simulink model "ARDroneControl"  (R2024a)
settings: Solver=ode1  StartTime=0.0  StopTime=inf  FixedStep=sampleTime  RelTol=1e-3  EnableMultiTasking=on
InitFcn:
  | run('/Users/usuario/Desktop/MEAer/TFM/End-end system/ARDroneSimulinkDevKit_V1.1 hover/wifiControl/DroneStream_tracking_init.m')
undefined symbols (not defined in the file): sampleTime, Standard_Devices, UDP_Protocol
libraries: sldrtlib x3, dspnetwork x3, aerolibanimutils x1
settings Model: ExtModeTrigDuration=100000  Creator=Paul  LastModifiedBy=usuario
settings SolverCC: AlgebraicLoopSolver=TrustRegion  AutoInsertRateTranBlk=on
settings DataIOCC: LimitDataPoints=on  SaveFormat=StructureWithTime  SignalLoggingSaveFormat=ModelDataLogs  ReturnWorkspaceOutputs=off  TimeSaveName=time
settings OptimizationCC: BlockReduction=off  OptimizeBlockIOStorage=off  BufferReuse=off  GlobalBufferReuse=off  ExpressionFolding=off  ExpressionDepthLimit=2147483647  LocalBlockOutputs=off  InitFltsAndDblsToZero=on  OptimizeDataStoreBuffers=off  BusAssignmentInplaceUpdate=off
settings DebuggingCC: UnderspecifiedInitializationDetection=Classic  MergeDetectMultiDrivingBlocksExec=none  SolverPrmCheckMsg=warning  FcnCallInpInsideContextMsg=warning  UnconnectedInputMsg=warning  UnconnectedOutputMsg=warning  UnconnectedLineMsg=warning  StateNameClashWarn=warning  SFUnexpectedBacktrackingDiag=warning  SFNoUnconditionalDefaultTransitionDiag=warning  SFExecutionAtInitializationDiag=none  ArithmeticOperatorsInVariantConditions=warning
settings HardwareCC: ProdBitPerLong=64  ProdHWDeviceType=Intel->x86-64 (Mac OS X)
settings ModelReferenceCC: EnableRefExpFcnMdlSchedulingChecks=on  PropagateSignalLabelsOutOfModel=off
settings SFSimCC: SimUseLocalCustomCode=off  CustomCodeUndefinedFunction=UseInterfaceOnly
settings RTWCC: Description=Simulink Desktop Real-Time  SystemTargetFile=sldrt.tlc  TemplateMakefile=sldrt.tmf  RTWUseLocalCustomCode=off  RTWCompilerOptimization=on  GPUComputeCapability=3.5
settings CodeAppCC: MaxIdLength=95  StateflowObjectComments=on
settings SimulinkDesktopRealTimeCC: TargetPreCompLibLocation=/Applications/MATLAB_R2017b.app/toolbox/sldrt/lib/maci64  TargetLangStandard=C89/C90 (ANSI)
settings ConfigComp: CovMetricSettings=dw  CovSaveCumulativeToWorkspaceVar=on  CovSaveSingleToWorkspaceVar=on  CovExternalEMLEnable=off

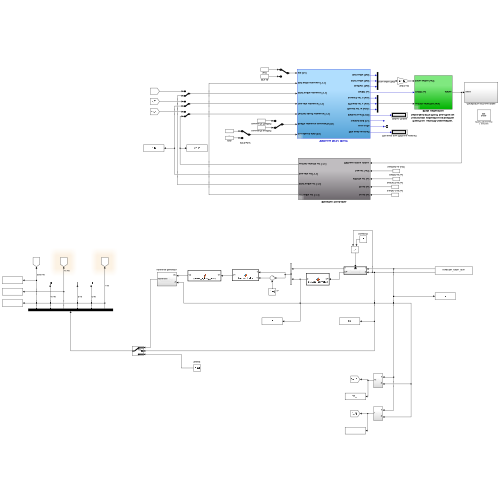
[thumbnail: Simulink's stored preview of the top-level diagram]
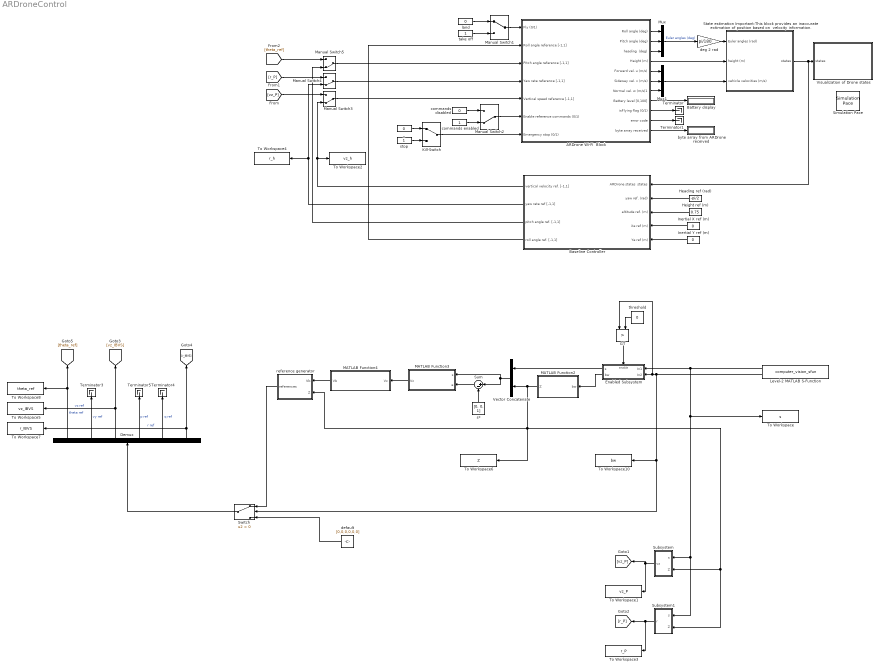
== system ARDroneControl ==
  ARDrone Wi-Fi  Block : Subsystem  AncestorBlock="ARBlocks/ARDrone Wi-Fi  Block"
  Baseline Controller : Subsystem  AncestorBlock=ARBlocks/Baseline Controller
  Battery display : Display
  Demux : Demux  Outputs=6
  Enabled Subsystem : Subsystem  TreatAsAtomicUnit=on
  GT : RelationalOperator  Operator=>  OutDataTypeStr=boolean  RndMeth=Simplest  InputSameDT=off
  Heading ref (rad) : Constant  Value=-pi/2
  Height ref (m) : Constant  Value=0.75
  Inertial X ref (m) : Constant  Value=0
  Inertial Y ref (m) : Constant  Value=0
  Kill-Switch : ManualSwitch
  Level-2 MATLAB S-Function : M-S-Function  FunctionName=computer_vision_sfun
  MATLAB Function2 : MATLAB Function  TreatAsAtomicUnit=on
  MATLAB Function3 : MATLAB Function  TreatAsAtomicUnit=on
  MATLAB Function4 : MATLAB Function  TreatAsAtomicUnit=on
  Manual Switch1 : ManualSwitch
  Manual Switch{2..5} (4 alike) : ManualSwitch  CurrentSetting=0
  Mux : Mux  Inputs=3
  Mux1 : Mux  Inputs=3
  Simulation Pace : aerolibanimutils/Simulation Pace  SimulationPace=1  SleepMode=MATLAB Thread  OutputPaceError=off  SampleTime=sampleTime
  "State estimation Important:This block provides an inaccurate extimation of position based on  velocity information. " : Subsystem  AncestorBlock=|
      | ARBlocks/Position estimation
      | Important:This block provides an 
      | inaccurate extimation of position 
      | based on  velocity information.
  Subsystem : Subsystem
  Subsystem1 : Subsystem
  Sum : Sum  Inputs=|+-
  Switch : Switch  Criteria=u2 > Threshold  SaturateOnIntegerOverflow=off  InputSameDT=off
  Terminator{,1,3..5} (5 alike) : Terminator
  To Workspace : ToWorkspace  VariableName=s  SaveFormat=Timeseries  SampleTime=-1
  To Workspace1 : ToWorkspace  VariableName=vz_P  SaveFormat=Timeseries  SampleTime=-1
  To Workspace10 : ToWorkspace  VariableName=bw  SaveFormat=Timeseries  SampleTime=-1
  To Workspace2 : ToWorkspace  VariableName=vz_h  SaveFormat=Timeseries  SampleTime=-1
  To Workspace3 : ToWorkspace  VariableName=r_P  SaveFormat=Timeseries  SampleTime=-1
  To Workspace4 : ToWorkspace  VariableName=r_h  SaveFormat=Timeseries  SampleTime=-1
  To Workspace5 : ToWorkspace  VariableName=vz_IBVS  SaveFormat=Timeseries  SampleTime=-1
  To Workspace6 : ToWorkspace  VariableName=Z  SaveFormat=Timeseries  SampleTime=-1
  To Workspace7 : ToWorkspace  VariableName=r_IBVS  SaveFormat=Timeseries  SampleTime=-1
  To Workspace8 : ToWorkspace  VariableName=theta_ref  SaveFormat=Timeseries  SampleTime=-1
  Vector Concatenate : Concatenate
  Visualization of Drone states : Subsystem
  _ : Constant  Value=0
  "byte array from ARDrone received " : Display
  commands disabled : Constant  Value=0
  commands enabled : Constant
  default : Constant  Value=[0,0,0,0,0,0]
  deg 2 rad : Gain  Gain=pi/180
  land : Constant  Value=0
  reference generator : Subsystem
  s* : Constant  Value=[0, 0, 1]
  stop : Constant
  take off : Constant
  threshold : Constant  Value=0
  wires:
  _/1 -> Kill-Switch/1
  stop/1 -> Kill-Switch/2
  land/1 -> Manual Switch1/1
  take off/1 -> Manual Switch1/2
  commands disabled/1 -> Manual Switch2/1
  commands enabled/1 -> Manual Switch2/2
  Manual Switch1/1 -> ARDrone Wi-Fi  Block/1(Fly (0/1))
  Manual Switch2/1 -> ARDrone Wi-Fi  Block/6(Enable reference commands (0/1))
  Kill-Switch/1 -> ARDrone Wi-Fi  Block/7(Emergency stop (0/1))
  ARDrone Wi-Fi  Block/1(Roll angle (deg)) -> Mux/1
  ARDrone Wi-Fi  Block/2(Pitch angle (deg)) -> Mux/2
  ARDrone Wi-Fi  Block/5(Forward vel. u (m/s)) -> Mux1/1
  ARDrone Wi-Fi  Block/6(Sideway vel. v (m/s)) -> Mux1/2
  ARDrone Wi-Fi  Block/7(Normal vel. w (m/s)1) -> Mux1/3
  Mux/1 -> deg 2 rad/1  "Euler angles (deg)"
  ARDrone Wi-Fi  Block/8(Battery level [0,100]) -> Battery display/1
  "State estimation Important:This block provides an inaccurate extimation of position based on  velocity information. "/1(states) -> Baseline Controller/1("ARDrone states  states "), Visualization of Drone states/1(states)
  deg 2 rad/1 -> "State estimation Important:This block provides an inaccurate extimation of position based on  velocity information. "/1(Euler angles (rad))
  Mux1/1 -> "State estimation Important:This block provides an inaccurate extimation of position based on  velocity information. "/3(vehicle velocities (m/s))
  ARDrone Wi-Fi  Block/3(heading  (deg)) -> Mux/3
  ARDrone Wi-Fi  Block/9(isFlying flag (0/1)) -> Terminator/1
  ARDrone Wi-Fi  Block/10(error code) -> Terminator1/1
  ARDrone Wi-Fi  Block/11(byte array received) -> "byte array from ARDrone received "/1
  ARDrone Wi-Fi  Block/4(Height (m)) -> "State estimation Important:This block provides an inaccurate extimation of position based on  velocity information. "/2(height (m))
  Heading ref (rad)/1 -> Baseline Controller/2(yaw ref. (rad))
  Inertial Y ref (m)/1 -> Baseline Controller/5(Ye ref (m))
  Inertial X ref (m)/1 -> Baseline Controller/4(Xe ref (m))
  Baseline Controller/4(roll angle ref. [-1,1]) -> ARDrone Wi-Fi  Block/2(Roll angle reference [-1,1])
  Height ref (m)/1 -> Baseline Controller/3(altitude ref. (m))
  s*/1 -> Sum/2
  Demux/4 -> Terminator5/1  "p ref"
  Demux/2 -> Terminator3/1  "vy ref"
  Sum/1 -> MATLAB Function3/2(e)
  Level-2 MATLAB S-Function/1 -> Subsystem1/1(s), Subsystem/1(s), To Workspace/1, Enabled Subsystem/1(In1)
  MATLAB Function2/1(Z) -> reference generator/2(Z), Subsystem/2(Z), Subsystem1/2(Z), To Workspace6/1, Vector Concatenate/2
  MATLAB Function3/1(Vc) -> MATLAB Function4/1(Vc)
  Demux/5 -> Terminator4/1  "q ref"
  Demux/3 -> To Workspace5/1, [vz_IBVS]  "vz ref"
  Demux/6 -> [r_IBVS], To Workspace7/1  "r ref"
  [vz_P] -> Manual Switch3/1
  [r_P] -> Manual Switch4/1
  Manual Switch4/1 -> ARDrone Wi-Fi  Block/4(Yaw rate reference [-1,1])
  Manual Switch3/1 -> ARDrone Wi-Fi  Block/5(Vertical speed reference [-1,1])
  Baseline Controller/1(vertical velocity ref. [-1,1]) -> Manual Switch3/2, To Workspace2/1
  Baseline Controller/2(yaw rate ref [-1,1]) -> Manual Switch4/2, To Workspace4/1
  Subsystem/1(vz) -> [vz_P], To Workspace1/1
  Subsystem1/1(r) -> To Workspace3/1, [r_P]
  Level-2 MATLAB S-Function/2 -> Enabled Subsystem/2(In2), GT/1, Switch/2, To Workspace10/1
  GT/1 -> Enabled Subsystem/Enable
  threshold/1 -> GT/2
  Switch/1 -> Demux/1
  default/1 -> Switch/3
  Enabled Subsystem/1(s) -> Vector Concatenate/1
  Enabled Subsystem/2(bw) -> MATLAB Function2/1(bw)
  Demux/1 -> To Workspace8/1, [theta_ref]  "theta ref"
  Manual Switch5/1 -> ARDrone Wi-Fi  Block/3(Pitch angle reference [-1,1])
  [theta_ref] -> Manual Switch5/1
  Baseline Controller/3(pitch angle ref. [-1,1]) -> Manual Switch5/2
  MATLAB Function4/1(Vb) -> reference generator/1(Vb)
  reference generator/1(references) -> Switch/1
  Vector Concatenate/1 -> Sum/1, MATLAB Function3/1(s)

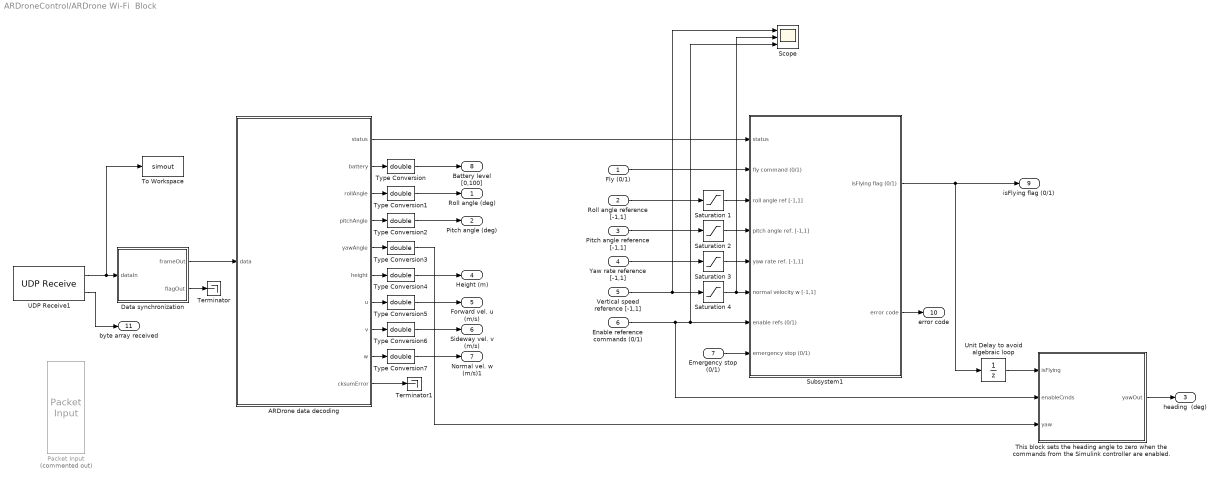
== system ARDroneControl/ARDrone Wi-Fi  Block ==
  Fly (0/1) : Inport
  Roll angle reference [-1,1] : Inport  Port=2
  Pitch angle reference [-1,1] : Inport  Port=3
  Yaw rate reference [-1,1] : Inport  Port=4
  Vertical speed reference [-1,1] : Inport  Port=5
  Enable reference commands (0/1) : Inport  Port=6
  Emergency stop (0/1) : Inport  Port=7
  ARDrone data decoding : MATLAB Function  TreatAsAtomicUnit=on
  "Data synchronization " : MATLAB Function  TreatAsAtomicUnit=on
  Packet Input : sldrtlib/Packet Input  Commented=on  SampleTime=sampleTime  MaxMissedTicks=100  ShowMissedTicks=off  YieldWhenWaiting=off  DrvName=Standard_Devices/UDP_Protocol  DrvAddress=5554  DrvOptions=[3232235777 5554]  PacketSize=500  DataTypes='500*uint8'  ShowReady=on  ShowError=off  PacketID=1  ByteOrder=1  ShowTimestamp=off
      settings: AttributesFormatString=UDP Protocol [5554]
  Saturation 1 : Saturate  UpperLimit=1  LowerLimit=-1
  Saturation 2 : Saturate  UpperLimit=1  LowerLimit=-1
  Saturation 3 : Saturate  UpperLimit=1  LowerLimit=-1
  Saturation 4 : Saturate  UpperLimit=1.5  LowerLimit=-1.5
  Scope : Scope  NumInputPorts=3
  Subsystem1 : Subsystem
  Terminator : Terminator
  Terminator1 : Terminator
  "This block sets the heading angle to zero when the commands from the Simulink controller are enabled. " : MATLAB Function  TreatAsAtomicUnit=on
  To Workspace : ToWorkspace  VariableName=simout  SampleTime=-1
  Type Conversion{,1..7} (8 alike) : DataTypeConversion  OutDataTypeStr=double  SaturateOnIntegerOverflow=off  RndMeth=Floor
  UDP Receive1 : dspnetwork/UDP Receive  localURL='0.0.0.0'  localPort=5554  remoteURL='192.168.1.1'  remotePort=-1  recvBufferSize=8192  dims=500  signalDatatype=uint8  isComplex=off  isVarSize=off  showBlockingTime=off  blockingTime=0  sampletime=sampleTime  blockPlatform=[]
  Unit Delay to avoid algebraic loop : UnitDelay  SampleTime=-1  HasFrameUpgradeWarning=on
  Roll angle (deg) : Outport  VectorParamsAs1DForOutWhenUnconnected=off
  Pitch angle (deg) : Outport  Port=2  VectorParamsAs1DForOutWhenUnconnected=off
  heading  (deg) : Outport  Port=3  VectorParamsAs1DForOutWhenUnconnected=off
  Height (m) : Outport  Port=4  VectorParamsAs1DForOutWhenUnconnected=off
  Forward vel. u (m/s) : Outport  Port=5  VectorParamsAs1DForOutWhenUnconnected=off
  Sideway vel. v (m/s) : Outport  Port=6  VectorParamsAs1DForOutWhenUnconnected=off
  Normal vel. w (m/s)1 : Outport  Port=7  VectorParamsAs1DForOutWhenUnconnected=off
  Battery level [0,100] : Outport  Port=8  VectorParamsAs1DForOutWhenUnconnected=off
  isFlying flag (0/1) : Outport  Port=9  VectorParamsAs1DForOutWhenUnconnected=off
  error code : Outport  Port=10  VectorParamsAs1DForOutWhenUnconnected=off
  byte array received : Outport  Port=11  VectorParamsAs1DForOutWhenUnconnected=off
  wires:
  Unit Delay to avoid algebraic loop/1 -> "This block sets the heading angle to zero when the commands from the Simulink controller are enabled. "/1(isFlying)
  "Data synchronization "/2(flagOut) -> Terminator/1
  Saturation 4/1 -> Scope/2, Subsystem1/6(normal velocity w [-1,1])
  Saturation 3/1 -> Subsystem1/5(yaw rate ref. [-1,1])
  Saturation 2/1 -> Subsystem1/4(pitch angle ref. [-1,1])
  Saturation 1/1 -> Subsystem1/3(roll angle ref [-1,1])
  Fly (0/1)/1 -> Subsystem1/2(fly command (0/1))
  "This block sets the heading angle to zero when the commands from the Simulink controller are enabled. "/1(yawOut) -> heading  (deg)/1
  Type Conversion3/1 -> "This block sets the heading angle to zero when the commands from the Simulink controller are enabled. "/3(yaw)
  Type Conversion7/1 -> Normal vel. w (m/s)1/1
  Type Conversion6/1 -> Sideway vel. v (m/s)/1
  Type Conversion5/1 -> Forward vel. u (m/s)/1
  Type Conversion4/1 -> Height (m)/1
  Type Conversion2/1 -> Pitch angle (deg)/1
  Type Conversion1/1 -> Roll angle (deg)/1
  Type Conversion/1 -> Battery level [0,100]/1
  ARDrone data decoding/10(cksumError) -> Terminator1/1
  Subsystem1/2(error code) -> error code/1
  Subsystem1/1(isFlying flag (0/1)) -> isFlying flag (0/1)/1, Unit Delay to avoid algebraic loop/1
  Emergency stop (0/1)/1 -> Subsystem1/8(emergency stop (0/1))
  Enable reference commands (0/1)/1 -> Scope/3, Subsystem1/7(enable refs (0/1)), "This block sets the heading angle to zero when the commands from the Simulink controller are enabled. "/2(enableCmds)
  Vertical speed reference [-1,1]/1 -> Scope/1, Saturation 4/1
  Yaw rate reference [-1,1]/1 -> Saturation 3/1
  Pitch angle reference [-1,1]/1 -> Saturation 2/1
  Roll angle reference [-1,1]/1 -> Saturation 1/1
  ARDrone data decoding/1(status) -> Subsystem1/1(status)
  UDP Receive1/2 -> byte array received/1
  ARDrone data decoding/9(w) -> Type Conversion7/1
  ARDrone data decoding/8(v) -> Type Conversion6/1
  ARDrone data decoding/7(u) -> Type Conversion5/1
  ARDrone data decoding/4(pitchAngle) -> Type Conversion2/1
  ARDrone data decoding/3(rollAngle) -> Type Conversion1/1
  ARDrone data decoding/6(height) -> Type Conversion4/1
  ARDrone data decoding/2(battery) -> Type Conversion/1
  ARDrone data decoding/5(yawAngle) -> Type Conversion3/1
  "Data synchronization "/1(frameOut) -> ARDrone data decoding/1(data)
  UDP Receive1/1 -> To Workspace/1, "Data synchronization "/1(dataIn)

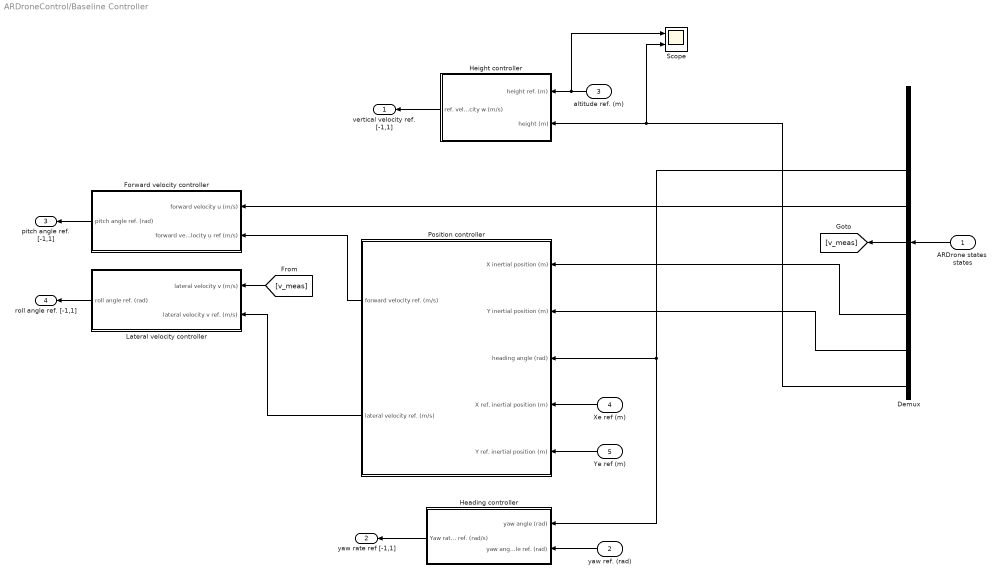
== system ARDroneControl/Baseline Controller ==
  "ARDrone states  states " : Inport
  yaw ref. (rad) : Inport  Port=2
  altitude ref. (m) : Inport  Port=3
  Xe ref (m) : Inport  Port=4
  Ye ref (m) : Inport  Port=5
  Demux : Demux  Outputs=9
  "Forward velocity controller " : Subsystem
  Heading controller : Subsystem
  "Height controller " : Subsystem
  Lateral velocity controller : Subsystem
  Position controller : Subsystem
  Scope : Scope  NumInputPorts=2
  vertical velocity ref. [-1,1] : Outport  VectorParamsAs1DForOutWhenUnconnected=off
  yaw rate ref [-1,1] : Outport  Port=2  VectorParamsAs1DForOutWhenUnconnected=off
  pitch angle ref. [-1,1] : Outport  Port=3  VectorParamsAs1DForOutWhenUnconnected=off
  roll angle ref. [-1,1] : Outport  Port=4  VectorParamsAs1DForOutWhenUnconnected=off
  wires:
  [v_meas] -> Lateral velocity controller/1(lateral velocity v (m/s))
  Demux/5 -> [v_meas]
  Position controller/2(lateral velocity ref. (m/s)) -> Lateral velocity controller/2(lateral velocity v ref. (m/s))
  Position controller/1(forward velocity ref. (m/s)) -> "Forward velocity controller "/2(forward velocity u ref (m/s))
  Ye ref (m)/1 -> Position controller/5(Y ref. inertial position (m))
  Xe ref (m)/1 -> Position controller/4(X ref. inertial position (m))
  Demux/8 -> Position controller/2(Y inertial position (m))
  Demux/7 -> Position controller/1(X inertial position (m))
  Heading controller/1(Yaw rate ref. (rad/s)) -> yaw rate ref [-1,1]/1
  yaw ref. (rad)/1 -> Heading controller/2(yaw angle ref. (rad))
  "Forward velocity controller "/1(pitch angle ref. (rad)) -> pitch angle ref. [-1,1]/1
  Demux/4 -> "Forward velocity controller "/1(forward velocity u (m/s))
  Lateral velocity controller/1(roll angle ref. (rad)) -> roll angle ref. [-1,1]/1
  "Height controller "/1(ref. velocity w (m/s)) -> vertical velocity ref. [-1,1]/1
  Demux/9 -> Scope/2, "Height controller "/2(height (m))
  altitude ref. (m)/1 -> Scope/1, "Height controller "/1(height ref. (m))
  Demux/3 -> Position controller/3(heading angle (rad)), Heading controller/1(yaw angle (rad))
  "ARDrone states  states "/1 -> Demux/1

== system ARDroneControl/Enabled Subsystem ==
  In1 : Inport
  In2 : Inport  Port=2
  Enable : EnablePort
  s : Outport
  bw : Outport  Port=2
  wires:
  In1/1 -> s/1
  In2/1 -> bw/1

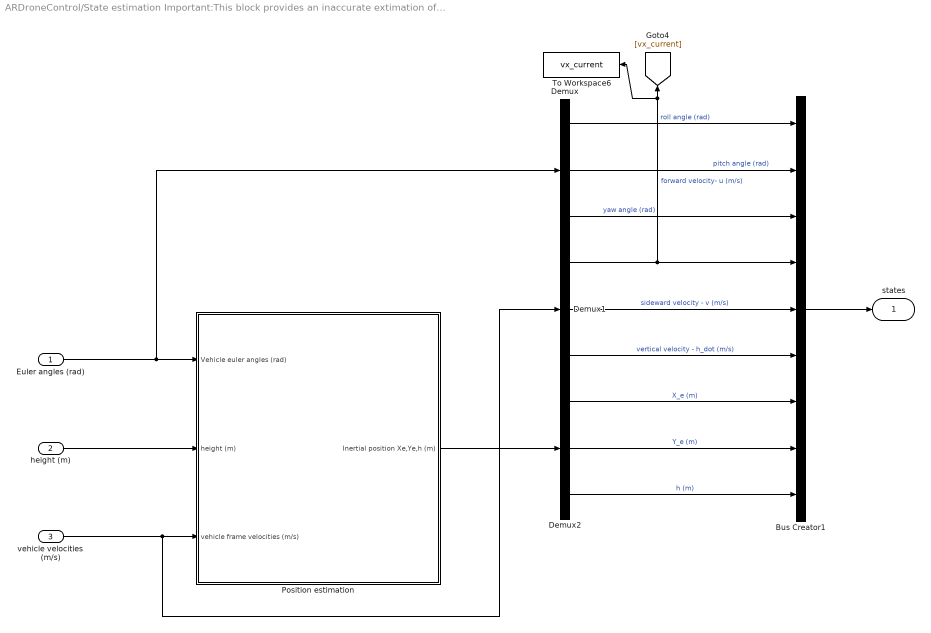
== system ARDroneControl/State estimation Important:This block provides an inaccurate extimation of position based on  velocity information.  ==
  Euler angles (rad) : Inport
  height (m) : Inport  Port=2
  vehicle velocities (m/s) : Inport  Port=3
  Bus Creator1 : BusCreator  Inputs=9
  Demux : Demux  Outputs=3
  Demux1 : Demux  Outputs=3
  Demux2 : Demux  Outputs=3
  Position estimation : Subsystem
  To Workspace6 : ToWorkspace  VariableName=vx_current  SaveFormat=Timeseries  SampleTime=-1
  states : Outport  VectorParamsAs1DForOutWhenUnconnected=off
  wires:
  height (m)/1 -> Position estimation/2(height (m))
  Bus Creator1/1 -> states/1
  Demux2/3 -> Bus Creator1/9  "h (m)"
  Demux2/2 -> Bus Creator1/8  "Y_e (m)"
  Demux2/1 -> Bus Creator1/7  "X_e (m)"
  Demux1/3 -> Bus Creator1/6  "vertical velocity - h_dot (m/s)"
  Demux1/2 -> Bus Creator1/5  "sideward velocity - v (m/s)"
  Demux1/1 -> Bus Creator1/4, To Workspace6/1, [vx_current]  "forward velocity- u (m/s)"
  Demux/3 -> Bus Creator1/3  "yaw angle (rad)"
  Demux/2 -> Bus Creator1/2  "pitch angle (rad)"
  Demux/1 -> Bus Creator1/1  "roll angle (rad)"
  Position estimation/1(Inertial position Xe,Ye,h (m)) -> Demux2/1
  Euler angles (rad)/1 -> Demux/1, Position estimation/1(Vehicle euler angles (rad))
  vehicle velocities (m/s)/1 -> Position estimation/3(vehicle frame velocities (m/s)), Demux1/1

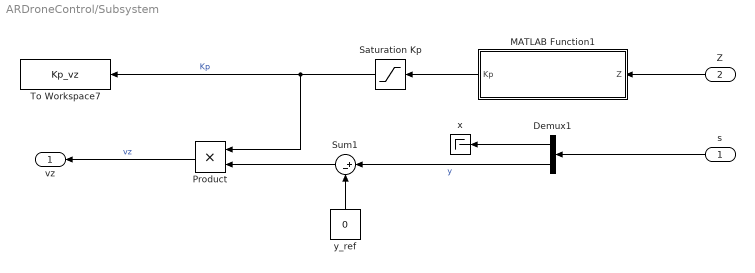
== system ARDroneControl/Subsystem ==
  s : Inport
  Z : Inport  Port=2
  Demux1 : Demux  Outputs=2
  MATLAB Function1 : MATLAB Function  TreatAsAtomicUnit=on
  Product : Product
  "Saturation Kp  " : Saturate  UpperLimit=-0.5
  Sum1 : Sum  Inputs=|+-
  To Workspace7 : ToWorkspace  VariableName=Kp_vz  SaveFormat=Timeseries  SampleTime=-1
  x : Terminator
  y_ref : Constant  Value=0
  vz : Outport
  wires:
  Sum1/1 -> Product/2
  Product/1 -> vz/1  "vz"
  s/1 -> Demux1/1
  y_ref/1 -> Sum1/2
  Demux1/1 -> x/1
  Demux1/2 -> Sum1/1  "y"
  MATLAB Function1/1(Kp) -> "Saturation Kp  "/1
  Z/1 -> MATLAB Function1/1(Z)
  "Saturation Kp  "/1 -> Product/1, To Workspace7/1  "Kp"

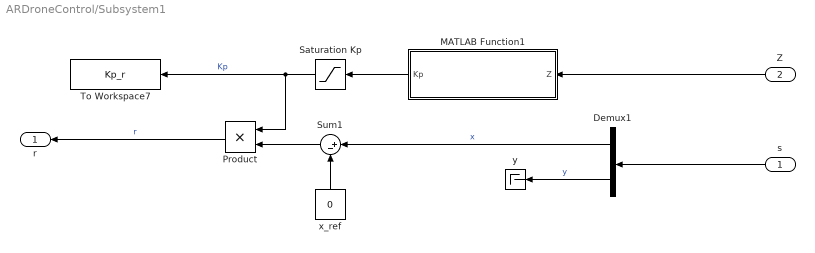
== system ARDroneControl/Subsystem1 ==
  s : Inport
  Z : Inport  Port=2
  Demux1 : Demux  Outputs=2
  MATLAB Function1 : MATLAB Function  TreatAsAtomicUnit=on
  Product : Product
  "Saturation Kp  " : Saturate  UpperLimit=0.008  LowerLimit=0.008
  Sum1 : Sum  Inputs=|+-
  To Workspace7 : ToWorkspace  VariableName=Kp_r  SaveFormat=Timeseries  SampleTime=-1
  x_ref : Constant  Value=0
  y : Terminator
  r : Outport
  wires:
  s/1 -> Demux1/1
  x_ref/1 -> Sum1/2
  Demux1/2 -> y/1  "y"
  Demux1/1 -> Sum1/1  "x"
  Sum1/1 -> Product/2
  MATLAB Function1/1(Kp) -> "Saturation Kp  "/1
  Z/1 -> MATLAB Function1/1(Z)
  Product/1 -> r/1  "r"
  "Saturation Kp  "/1 -> Product/1, To Workspace7/1  "Kp"

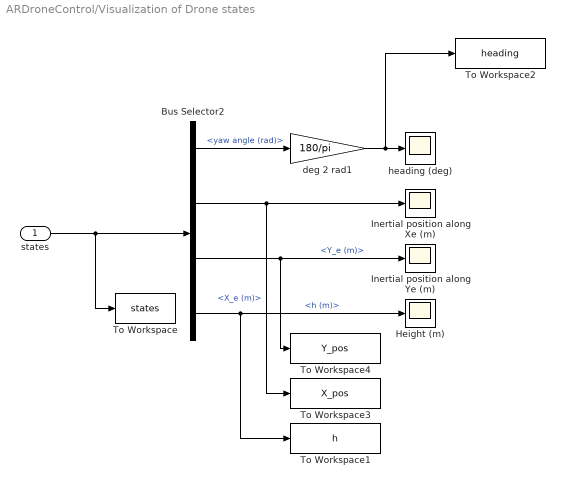
== system ARDroneControl/Visualization of Drone states ==
  states : Inport
  Bus Selector2 : BusSelector  OutputSignals=yaw angle (rad),X_e (m),Y_e (m),h (m)
  Height (m) : Scope
  Inertial position along Xe (m) : Scope
  Inertial position along Ye (m) : Scope
  To Workspace : ToWorkspace  VariableName=states  SaveFormat=Structure With Time  SampleTime=-1
  To Workspace1 : ToWorkspace  VariableName=h  SaveFormat=Timeseries  SampleTime=-1
  To Workspace2 : ToWorkspace  VariableName=heading  SaveFormat=Timeseries  SampleTime=-1
  To Workspace3 : ToWorkspace  VariableName=X_pos  SaveFormat=Timeseries  SampleTime=-1
  To Workspace4 : ToWorkspace  VariableName=Y_pos  SaveFormat=Timeseries  SampleTime=-1
  deg 2 rad1 : Gain  Gain=180/pi
  heading (deg) : Scope
  wires:
  states/1 -> To Workspace/1, Bus Selector2/1
  Bus Selector2/1 -> deg 2 rad1/1  "<yaw angle (rad)>"
  Bus Selector2/2 -> Inertial position along Xe (m)/1, To Workspace3/1  "<X_e (m)>"
  Bus Selector2/3 -> Inertial position along Ye (m)/1, To Workspace4/1  "<Y_e (m)>"
  Bus Selector2/4 -> Height (m)/1, To Workspace1/1  "<h (m)>"
  deg 2 rad1/1 -> To Workspace2/1, heading (deg)/1

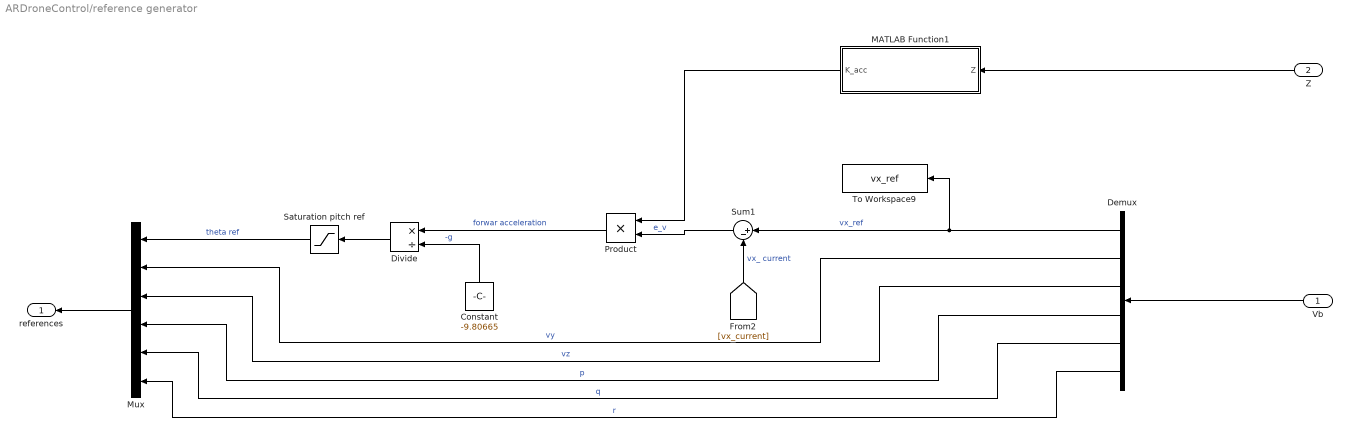
== system ARDroneControl/reference generator ==
  Vb : Inport
  Z : Inport  Port=2
  Constant : Constant  Value=-9.80665
  Demux : Demux  Outputs=6
  Divide : Product  Inputs=*/
  MATLAB Function1 : MATLAB Function  TreatAsAtomicUnit=on
  Mux : Mux  Inputs=6
  Product : Product
  Saturation pitch ref : Saturate  UpperLimit=0.052  LowerLimit=-0.052
  Sum1 : Sum  Inputs=|+-
  To Workspace9 : ToWorkspace  VariableName=vx_ref  SaveFormat=Timeseries  SampleTime=-1
  references : Outport  VectorParamsAs1DForOutWhenUnconnected=off
  wires:
  [vx_current] -> Sum1/2  "vx_ current"
  Constant/1 -> Divide/2  "-g"
  Divide/1 -> Saturation pitch ref/1
  Vb/1 -> Demux/1
  Demux/1 -> To Workspace9/1, Sum1/1  "vx_ref"
  Saturation pitch ref/1 -> Mux/1  "theta ref"
  Demux/2 -> Mux/2  "vy"
  Demux/3 -> Mux/3  "vz"
  Demux/4 -> Mux/4  "p"
  Demux/5 -> Mux/5  "q"
  Demux/6 -> Mux/6  "r"
  Mux/1 -> references/1
  Product/1 -> Divide/1  "forwar acceleration"
  Sum1/1 -> Product/2  "e_v"
  MATLAB Function1/1(K_acc) -> Product/1
  Z/1 -> MATLAB Function1/1(Z)

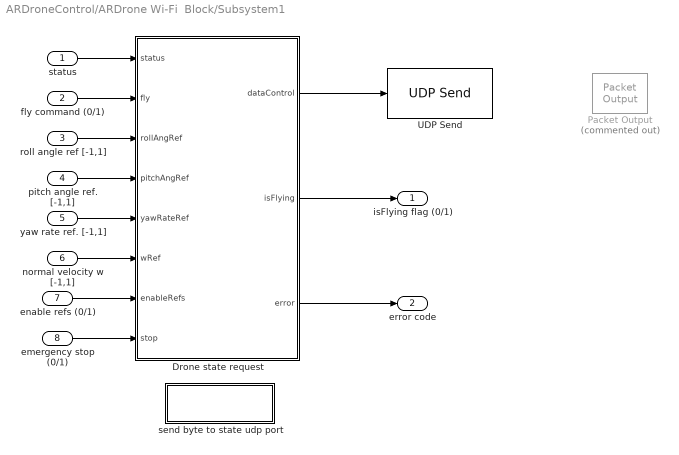
== system ARDroneControl/ARDrone Wi-Fi  Block/Subsystem1 ==
  status : Inport
  fly command (0/1) : Inport  Port=2
  roll angle ref [-1,1] : Inport  Port=3
  pitch angle ref. [-1,1] : Inport  Port=4
  yaw rate ref. [-1,1] : Inport  Port=5
  normal velocity w [-1,1] : Inport  Port=6
  enable refs (0/1) : Inport  Port=7
  emergency stop (0/1) : Inport  Port=8
  Drone state request : MATLAB Function  TreatAsAtomicUnit=on  SystemSampleTime=sampleTime
  Packet Output : sldrtlib/Packet Output  Commented=on  SampleTime=sampleTime*7  MaxMissedTicks=100  ShowMissedTicks=off  YieldWhenWaiting=off  DrvName=Standard_Devices/UDP_Protocol  DrvAddress=5556  DrvOptions=[3232235777 5556]  PacketSize=150  DataTypes='150*uint8'  ShowReady=off  ShowError=off  PacketID=1  ByteOrder=1  InitialValue=[]  FinalValue=[]
      settings: AttributesFormatString=UDP Protocol [5556]
  UDP Send : dspnetwork/UDP Send  remoteURL='192.168.1.1'  remotePort=5556  localURL='0.0.0.0'  localPortSource=Specify via dialog  localPort=5556  sendBufferSize=8192  sampletime=-1  blockPlatform=[]  separateLengthPort=0
  "send byte to state udp port " : Subsystem
  isFlying flag (0/1) : Outport  VectorParamsAs1DForOutWhenUnconnected=off
  error code : Outport  Port=2  VectorParamsAs1DForOutWhenUnconnected=off
  wires:
  Drone state request/3(error) -> error code/1
  emergency stop (0/1)/1 -> Drone state request/8(stop)
  enable refs (0/1)/1 -> Drone state request/7(enableRefs)
  normal velocity w [-1,1]/1 -> Drone state request/6(wRef)
  yaw rate ref. [-1,1]/1 -> Drone state request/5(yawRateRef)
  roll angle ref [-1,1]/1 -> Drone state request/3(rollAngRef)
  Drone state request/2(isFlying) -> isFlying flag (0/1)/1
  status/1 -> Drone state request/1(status)
  pitch angle ref. [-1,1]/1 -> Drone state request/4(pitchAngRef)
  fly command (0/1)/1 -> Drone state request/2(fly)
  Drone state request/1(dataControl) -> UDP Send/1

== system ARDroneControl/Baseline Controller/Forward velocity controller  ==
  forward velocity u (m/s) : Inport
  forward velocity u ref (m/s) : Inport  Port=2
  Gain : Gain  Gain=-0.5*1/2
  Sum2 : Sum  Inputs=|-+
  pitch angle ref. (rad) : Outport  VectorParamsAs1DForOutWhenUnconnected=off
  wires:
  forward velocity u ref (m/s)/1 -> Sum2/2
  Gain/1 -> pitch angle ref. (rad)/1
  Sum2/1 -> Gain/1
  forward velocity u (m/s)/1 -> Sum2/1

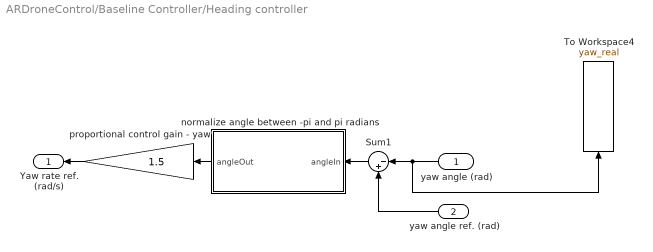
== system ARDroneControl/Baseline Controller/Heading controller ==
  yaw angle (rad) : Inport
  yaw angle ref. (rad) : Inport  Port=2
  Sum1 : Sum  Inputs=|-+
  To Workspace4 : ToWorkspace  VariableName=yaw_real  SaveFormat=Timeseries  SampleTime=-1
  normalize angle between -pi and pi radians : MATLAB Function  TreatAsAtomicUnit=on
  proportional control gain - yaw : Gain  Gain=1.5
  Yaw rate ref. (rad/s) : Outport  VectorParamsAs1DForOutWhenUnconnected=off
  wires:
  yaw angle ref. (rad)/1 -> Sum1/2
  proportional control gain - yaw/1 -> Yaw rate ref. (rad/s)/1
  yaw angle (rad)/1 -> To Workspace4/1, Sum1/1
  normalize angle between -pi and pi radians/1(angleOut) -> proportional control gain - yaw/1
  Sum1/1 -> normalize angle between -pi and pi radians/1(angleIn)

== system ARDroneControl/Baseline Controller/Height controller  ==
  height ref. (m) : Inport
  height (m) : Inport  Port=2
  Sum3 : Sum  Inputs=|-+
  proportional control gain : Gain  Gain=0.5
  ref. velocity w (m/s) : Outport  VectorParamsAs1DForOutWhenUnconnected=off
  wires:
  height ref. (m)/1 -> Sum3/2
  height (m)/1 -> Sum3/1
  Sum3/1 -> proportional control gain/1
  proportional control gain/1 -> ref. velocity w (m/s)/1

== system ARDroneControl/Baseline Controller/Lateral velocity controller ==
  lateral velocity v (m/s) : Inport
  lateral velocity v ref. (m/s) : Inport  Port=2
  Gain1 : Gain  Gain=0.4
  Sum5 : Sum  Inputs=|-+
  roll angle ref. (rad) : Outport  VectorParamsAs1DForOutWhenUnconnected=off
  wires:
  lateral velocity v ref. (m/s)/1 -> Sum5/2
  Gain1/1 -> roll angle ref. (rad)/1
  Sum5/1 -> Gain1/1
  lateral velocity v (m/s)/1 -> Sum5/1

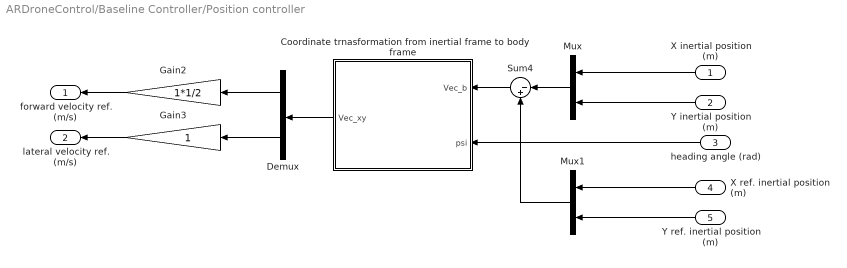
== system ARDroneControl/Baseline Controller/Position controller ==
  X inertial position (m) : Inport
  Y inertial position (m) : Inport  Port=2
  heading angle (rad) : Inport  Port=3
  X ref. inertial position (m) : Inport  Port=4
  Y ref. inertial position (m) : Inport  Port=5
  "Coordinate trnasformation from inertial frame to body frame " : MATLAB Function  TreatAsAtomicUnit=on
  Demux : Demux  Outputs=2
  Gain2 : Gain  Gain=1*1/2
  Gain3 : Gain
  Mux : Mux  Inputs=2
  Mux1 : Mux  Inputs=2
  Sum4 : Sum  Inputs=|-+
  forward velocity ref. (m/s) : Outport  VectorParamsAs1DForOutWhenUnconnected=off
  lateral velocity ref. (m/s) : Outport  Port=2  VectorParamsAs1DForOutWhenUnconnected=off
  wires:
  Gain3/1 -> lateral velocity ref. (m/s)/1
  Demux/2 -> Gain3/1
  Demux/1 -> Gain2/1
  Y ref. inertial position (m)/1 -> Mux1/2
  X ref. inertial position (m)/1 -> Mux1/1
  Mux/1 -> Sum4/1
  X inertial position (m)/1 -> Mux/1
  Y inertial position (m)/1 -> Mux/2
  Sum4/1 -> "Coordinate trnasformation from inertial frame to body frame "/1(Vec_b)
  Mux1/1 -> Sum4/2
  "Coordinate trnasformation from inertial frame to body frame "/1(Vec_xy) -> Demux/1
  heading angle (rad)/1 -> "Coordinate trnasformation from inertial frame to body frame "/2(psi)
  Gain2/1 -> forward velocity ref. (m/s)/1

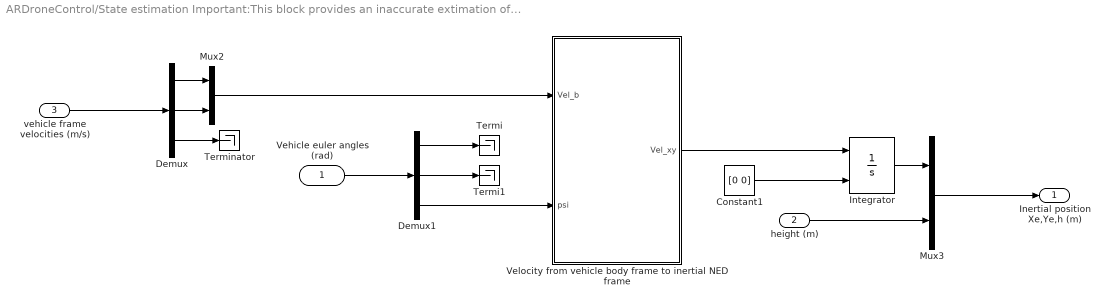
== system ARDroneControl/State estimation Important:This block provides an inaccurate extimation of position based on  velocity information. /Position estimation ==
  Vehicle euler angles (rad) : Inport
  height (m) : Inport  Port=2
  vehicle frame velocities (m/s) : Inport  Port=3
  Constant1 : Constant  Value=[0 0]
  Demux : Demux  Outputs=3
  Demux1 : Demux  Outputs=3
  Integrator : Integrator  InitialConditionSource=external
  Mux2 : Mux  Inputs=2
  Mux3 : Mux  Inputs=2
  Termi : Terminator
  Termi1 : Terminator
  Terminator : Terminator
  Velocity from vehicle body frame to inertial NED  frame : MATLAB Function  TreatAsAtomicUnit=on
  Inertial position Xe,Ye,h (m) : Outport  VectorParamsAs1DForOutWhenUnconnected=off
  wires:
  Mux3/1 -> Inertial position Xe,Ye,h (m)/1
  height (m)/1 -> Mux3/2
  Vehicle euler angles (rad)/1 -> Demux1/1
  vehicle frame velocities (m/s)/1 -> Demux/1
  Demux1/3 -> Velocity from vehicle body frame to inertial NED  frame/2(psi)
  Integrator/1 -> Mux3/1
  Constant1/1 -> Integrator/2
  Velocity from vehicle body frame to inertial NED  frame/1(Vel_xy) -> Integrator/1
  Demux1/2 -> Termi1/1
  Demux1/1 -> Termi/1
  Mux2/1 -> Velocity from vehicle body frame to inertial NED  frame/1(Vel_b)
  Demux/1 -> Mux2/1
  Demux/2 -> Mux2/2
  Demux/3 -> Terminator/1

== system ARDroneControl/ARDrone Wi-Fi  Block/Subsystem1/send byte to state udp port  ==
  Constant : Constant  Value=[1 ;13]  OutDataTypeStr=uint8
  Packet Output : sldrtlib/Packet Output  Commented=on  SampleTime=sampleTime*10  MaxMissedTicks=100  ShowMissedTicks=off  YieldWhenWaiting=off  DrvName=Standard_Devices/UDP_Protocol  DrvAddress=5554  DrvOptions=[3232235777 5554]  PacketSize=2  DataTypes='2*uint8'  ShowReady=off  ShowError=off  PacketID=1  ByteOrder=1  InitialValue=[]  FinalValue=[]
      settings: AttributesFormatString=UDP Protocol [5554]
  Rate Transition : RateTransition
  UDP Send : dspnetwork/UDP Send  remoteURL='192.168.1.1'  remotePort=5554  localURL='0.0.0.0'  localPortSource=Specify via dialog  localPort=5554  sendBufferSize=8192  sampletime=-1  blockPlatform=[]  separateLengthPort=0
  wires:
  Constant/1 -> Rate Transition/1
  Rate Transition/1 -> UDP Send/1

== matlab function ARDroneControl/MATLAB Function4 ==
  data: Vc input; Vb output
function Vb = camera_2_body_frame(Vc)

theta_x = pi/2;
theta_y = pi/2;

t = [0, 0, 0.197]; % distance camera centre of mass

Rx = [1, 0, 0;
         0, cos(theta_x), -sin(theta_x);
         0, sin(theta_x), cos(theta_x)];

Ry = [cos(theta_y), 0, sin(theta_y);
           0, 1, 0;
           -sin(theta_y), 0, cos(theta_y)];

R = Rx*Ry;

%Skew-symmetric matrix
t_skew = [0,-t(3),0;t(3),0,0;0,0,0];

T = [R, t_skew*R;
     zeros(3,3), R];

Vb = T*Vc;

== matlab function ARDroneControl/Subsystem/MATLAB Function1 ==
  data: Z input; Kp output
function Kp = altitude_decay_gain(Z)

    M = -0.8;
    Z_star = 0;

    sigma = sqrt(((-0.5)^1)/log(0.9));

    Kp = M*(1-exp(-0.5*((Z-Z_star)/sigma)^2));

end

== matlab function ARDroneControl/reference generator/MATLAB Function1 ==
  data: Z input; K_acc output
function K_acc = forward_acceleration(Z)

    M = 1;
    Z_star = 1;

    sigma = sqrt(((-0.5)^3)/log(0.85));

    K_acc = M*(1-exp(-0.5*((Z-Z_star)/sigma)^2));

end

== matlab function ARDroneControl/Baseline Controller/Position controller/Coordinate trnasformation from inertial frame to body frame  ==
  data: Vec_b input; Vec_xy output; psi input
function Vec_xy  = fcn(Vec_b , psi)
%#codegen
T = [cos(psi) sin(psi) ; -sin(psi) cos(psi)] ; 
Vec_xy = T*Vec_b(1:2,1);

== matlab function ARDroneControl/ARDrone Wi-Fi  Block/Subsystem1/Drone state request ==
  data: status input; fly input; rollAngRef input; pitchAngRef input; yawRateRef input; wRef input; enableRefs input; dataControl output; isFlying output; stop input; error output
function [dataControl, isFlying, error] = fcn( status, fly, rollAngRef, pitchAngRef, yawRateRef, wRef, enableRefs, stop)
%#codegen

% Persistent variables.
persistent SequenceNumber ;

% Initialization of persistent variables at first time step. 

if isempty(SequenceNumber)
    SequenceNumber = 1 ;
end



% Error code / No error: 0
error=0;

% Boolean of flying status / Flying: 1
isFlying = status(32) ;

% Byte array of size 150 to be sent to the drone.
strOut = uint8(zeros(150,1)) ;

% String that coontains a variable size command. 
% cmd is concatenated with previous commands at each sample
cmd = '';

% At first time step and every 100 time steps, data is requested.
if (SequenceNumber <=1 || mod(SequenceNumber, 100) ==0 )
    SequenceNumber = SequenceNumber+1; 
    strCmd = getString(SequenceNumber) ;
    cmd = ['AT*CONFIG=' strCmd ',"general:navdata_demo","TRUE"' char(13)];
    
end

SequenceNumber = SequenceNumber+1;
strCmd = getString(SequenceNumber) ;
cmd = [cmd 'AT*COMWDG=' strCmd char(13)];


if stop ==1 % Emergency stop
   cmd = ['AT*REF=' strCmd ',290717952' char(13)] ; 
    
else % Not emergency stop
    
    if SequenceNumber >20 && SequenceNumber <22
        
        % Trim vehicle state estimation / angles set to zero
        SequenceNumber =SequenceNumber+1;
        strCmd = getString(SequenceNumber) ;
        cmd = [cmd 'AT*FTRIM=' strCmd char(13)] ;
        
    elseif SequenceNumber >=22 && SequenceNumber <25
        cmd = [cmd 'AT*CONFIG=' strCmd '"conrol:altitude_max","100000"' char(13)] ;
        
        
    elseif SequenceNumber >=25
        
        if ( fly == 1  )
            
            if (isFlying ==0)
                
                SequenceNumber =SequenceNumber+1;
                strCmd = getString(SequenceNumber) ;
                cmd = [cmd 'AT*REF=' strCmd ',290718208' char(13)] ;
            
            elseif isFlying==1 && enableRefs==1
                
                SequenceNumber =SequenceNumber+1;
                strCmd = getString(SequenceNumber) ;
                      
                cmd = [cmd 'AT*PCMD=' strCmd ',1,'] ;
                 
                aux = double (float2IEEE754 (rollAngRef) )  ;
                strAux = getString(abs(aux)) ; 
                if rollAngRef<0
                   strAux = [char(45) strAux] ; 
                end
                cmd = [cmd strAux ','];
                      
               aux = double (float2IEEE754 (pitchAngRef) ) ;
               strAux = getString(abs(aux)) ; 
               if pitchAngRef<0
                    strAux = [char(45) strAux] ; 
               end
               cmd = [cmd strAux ','];
                      
               aux =  double(float2IEEE754 (wRef)) ;
               strAux = getString(abs(aux)) ; 
               if wRef<0
                    strAux = [char(45) strAux] ; 
               end
               cmd = [cmd strAux ','];
                      
                      
               aux =  double (float2IEEE754 (yawRateRef) ) ;
               strAux = getString(abs(aux)) ; 
               if yawRateRef <0
                     error=2; 
                     strAux = [char(45) strAux] ; 
               end
               cmd = [cmd strAux char(13)];
               
                
            end
            
            
        elseif ( fly==0 )
                
               if isFlying ==1
                    SequenceNumber =SequenceNumber+1;
                    strCmd = getString(SequenceNumber) ;
                    cmd = [cmd 'AT*REF=' strCmd ',290717696' char(13)] ;
                    
              end
        end
        
    end
    
    
    
end

% cmd must contain less than 150 bytes. 
if (length(cmd)<150)
    strOut(1:length(cmd)) = cmd ;
else
    error =1; 
end

dataControl = strOut;

end


%% My str2num function that allows for code generation
function [ strOut] = getString( a )
d=1;

if (a<10)
    d=1;
end

if (a >=10 && a <100)
    d=2;
end

if (a >=100 && a <1000)
    d=3;
end

if (a >=1000 && a <10000)
    d=4;
end

if (a >=10000 && a <100000)
    d=5;
end

if (a >=100000 && a <1000000)
    d=6;
end

if (a >=1000000 && a <10000000)
    d=7;
end

if (a >=10000000 && a <100000000)
    d=8;
end

if (a >=100000000 && a <1000000000)
    d=9;
end

if (a >=1000000000 && a <10000000000)
    d=10;
end

if (a >=10000000000 )
    d=11;
end



digit = uint8(zeros(1,d)) ;
resTotal = 0;
%d = length(a) ;
for k=1:d
    
    res1 = mod(a,10^k)/(10^(k-1)) ;
    %( mod(a,10*k) - resTotal)/(10*k) ;
    
    digit(d-k+1) = char(48 + res1);
    resTotal = (10^(k-1))*res1 +resTotal;
    
end

strOut = char(digit) ;


end

%% Function to obtain a IEEE754 representation of a float number
function [ iVal ] = float2IEEE754( fVal )

binData = dec2bin(typecast (single(fVal), 'uint8'),8);

binData2 =[ binData(4,:) binData(3,:) binData(2,:) binData(1,:)];
iVal =0; 
for k=32:-1:1
    
    if (binData2(k) =='1')
        bit = 1;
    else
        bit =0;
    end
    
    if k == 1
        iVal = iVal - bit*2^(31);
    else
        iVal = iVal + bit*2^(32-k) ; 
    end
    
end

iVal = int32(iVal);

end

== matlab function ARDroneControl/ARDrone Wi-Fi  Block/ARDrone data decoding ==
  data: status output; battery output; rollAngle output; pitchAngle output; data input; yawAngle output; height output; u output; v output; w output; cksumError output
function [ status, battery,  rollAngle, pitchAngle, yawAngle, height, u,v,w , cksumError ]= fcn(data)
%#codegen

% Checksum array. cksum(1) contains the computed checksum, cksum(2)
% contains the checksum sent by the ARDrone. 
cksum = [0 0 ]; 

% Previous value of height 
persistent hPrev ; 
% Previous data packet
persistent dataPrev ; 

% Initialization of persistent variables
if isempty(hPrev)
    hPrev=0 ; 
end

if isempty(dataPrev)
    dataPrev = uint8(zeros(496,1)) ;
end

% Computing checksum
cksum(1) =  sum(double(data(1:end-8))) +442; 
% Checksum given by the drone
cksum(2) = double(data(end-3)) + double(data(end-2))*256 +  double(data(end-1))*256^2 + double(data(end))*256^3 ; 
% Checksum error
cksumError = abs(cksum(1)-cksum(2));
%% Change the following if statement to ensure that the data checksum is valid 
%if (data(15) == 148 && cksumError==0 )
if (data(15) == 148  )
    dataPrev = data; 
else
    data = dataPrev; 
end

% Converting bytes to drone information
status = getDroneState(data(1:4));
battery = decode(data(21:24),1); % unit: deg
pitchAngle = decode(data(25:28),0)/1000; % unit: deg
rollAngle = decode(data(29:32),0)/1000; % unit: deg
yawAngle = decode(data(33:36),0)/1000; % unit: deg
height = double(decode(data(37:40),1))/1000; % unit: deg
u = decode(data(41:44),0)/1000; % unit: m/s
v = decode(data(45:48),0)/1000; % unit: m/s
w = decode(data(49:52),0)/1000; % unit: m/s



if (status(32) ==1 && height< 0.2   )
    height = hPrev;
elseif status(32)==1 
    hPrev= height; 
end
  
    
end


function res = decode(input, mark)
% if mark = 1; then output a int
% else output the float value which is defined by SDK description.
% the input is an array (1*4) 
% e.g. : NDS(Battery_OS:Battery_OS+data_length-1)
%    hex_value = dec2hex(input);
%    hex_value = [hex_value(4,:),hex_value(3,:),hex_value(2,:),hex_value(1,:)];
    if mark ==1
        res = typecast(input,'uint32')%hex2num(hex_value);
    else
        res = typecast(input,'single'); %res = typecast(uint32(hex2dec(hex_value)),'single');
    end
    res = res(1);
end

function bin = getDroneState(input)
    bin = zeros(32,1); 
    hex = dec2hex(input);
    % put the hex_value in the order [31, 30......0]
    hex = [hex(4,:),hex(3,:),hex(2,:),hex(1,:)];
for i=1:length(hex)
    if hex(i)=='F'
        bin((i*4)-3:i*4)=[1 1 1 1];
    elseif hex(i)=='E'
        bin((i*4)-3:i*4)=[1 1 1 0];
    elseif hex(i)=='D'
        bin((i*4)-3:i*4)=[1 1 0 1];
    elseif hex(i)=='C'
        bin((i*4)-3:i*4)=[1 1 0 0];
    elseif hex(i)=='B'
        bin((i*4)-3:i*4)=[1 0 1 1];
    elseif hex(i)=='A'
        bin((i*4)-3:i*4)=[1 0 1 0];
    elseif hex(i)=='9'
        bin((i*4)-3:i*4)=[1 0 0 1];
    elseif hex(i)=='8'
        bin((i*4)-3:i*4)=[1 0 0 0];
    elseif hex(i)=='7'
        bin((i*4)-3:i*4)=[0 1 1 1];
    elseif hex(i)=='6'
        bin((i*4)-3:i*4)=[0 1 1 0];
    elseif hex(i)=='5'
        bin((i*4)-3:i*4)=[0 1 0 1];
    elseif hex(i)=='4'
        bin((i*4)-3:i*4)=[0 1 0 0];
    elseif hex(i)=='3'
        bin((i*4)-3:i*4)=[0 0 1 1];
    elseif hex(i)=='2'
        bin((i*4)-3:i*4)=[0 0 1 0];
    elseif hex(i)=='1'
        bin((i*4)-3:i*4)=[0 0 0 1];
    elseif hex(i)=='0'
        bin((i*4)-3:i*4)=[0 0 0 0];
    end
end

end

== matlab function ARDroneControl/ARDrone Wi-Fi  Block/Data synchronization  ==
  data: dataIn input; frameOut output; flagOut output
function [frameOut,flagOut]  = fcn(dataIn)
%#eml
%% Author: David Escobar Sanabria
%  Description: This function synchronizes data coming from the flight computer
%  computer. 
%  frameOut: Organized frame
%  frameIn: sequence of bytes not sync.
persistent frame; 
persistent lastFrame; 
persistent count; 
persistent countHeader; 
persistent countBuffer; 
persistent buffer; 

%% Size of byte array containing the data
sizePayload= 496;

%% Size of the array read each time step
nBytes = 500 ;%size(dataIn,1); 


%%%%%%%%%%%%%%%%%%%%%%%%%%%%%%%%%%%%%%%%%%%%%%%%%%%%%%%
%% Initialization of presistent variables
if isempty(buffer)
    buffer=uint8(zeros(1024,1));
end

if isempty(countBuffer)
    countBuffer=0;
end


if isempty(frame)
    frame=uint8(zeros(sizePayload,1));
end

if isempty(lastFrame)
    lastFrame=uint8(zeros(sizePayload,1));
end


if isempty(count)
    count=0;
end

if isempty(countHeader)
    countHeader=0;
end
%%%%%%%%%%%%%%%%%%%%%%%%%%%%%%%%%%%%%%%%%%%%%%%%%%%%%%%

%% Filling the buffer
buffer(countBuffer+1:countBuffer+nBytes) = dataIn;

bytesToRead = countBuffer+nBytes; 

%%%%%%%%%%%%%%%%%%%%%%%%%%%%%%%%%%%%%%%%%%%%%%%%%%%%%%%
%% Reading buffer

for k=1:bytesToRead    
    if(countHeader==4 && count<sizePayload)
        bytesLeft = sizePayload-count;
        frame(count+1:sizePayload) = buffer(k:k+bytesLeft-1);
        count = sizePayload;
        countBuffer = bytesToRead-bytesLeft ;
        buffer(1:countBuffer) = buffer(k+bytesLeft:bytesToRead);
        break;
        
    end
    
    if(countHeader==3 && buffer(k)==85)
        
        countHeader=4;
 
        if(bytesToRead-k > sizePayload)
            count =sizePayload;  
            frame(1:count) = buffer(k+1:k+sizePayload);  
            countBuffer =bytesToRead-k-sizePayload ; 
            buffer(1:countBuffer) = buffer(k+sizePayload+1:bytesToRead);
        else
            
            count =bytesToRead-k;
            if count > 0          
                frame(1:count) = buffer(k+1:bytesToRead);  
            end
            countBuffer = 0; 
            
        end
        
        break;
    end
    
    if(countHeader==2 && buffer(k)==102)
        countHeader=3;
    end
    
    if(countHeader==1 && buffer(k)==119)
        countHeader=2;
    end
       
    if(countHeader==0 && buffer(k)==136)
        countHeader=1;
    end

end

if count==sizePayload 
     frameOut = frame;
     flagOut = 1; 
     lastFrame = frame;
     frame=uint8(zeros(sizePayload,1));
     count=0;
     countHeader=0;
     
else % In case the buffer does not have an entire payload
    frameOut = lastFrame;
    flagOut = 0; 
end

== matlab function ARDroneControl/ARDrone Wi-Fi  Block/This block sets the heading angle to zero when the commands from the Simulink controller are enabled.  ==
  data: isFlying input; enableCmds input; yawOut output; yaw input
% Description: This function zeroes out the heading angle once the commands
% are enabled. 
function yawOut = fcn(isFlying,enableCmds,yaw)
%#codegen

yawOut = yaw; 
persistent yaw0 ; 
persistent mode ; 

if isempty (yaw0)
yaw0 = 0; 
end


if isempty (mode)
mode=0; 
end

if isFlying ==1 && enableCmds==1    
    yawOut = yaw - yaw0; 
    mode =1; 
elseif isFlying ==1 && mode ==0
    yaw0 = yaw; 
end


yawOut = mod(yawOut, 360) ;
if yawOut > 180
    yawOut = -360 + yawOut ; 
end

== matlab function ARDroneControl/State estimation Important:This block provides an inaccurate extimation of position based on  velocity information. /Position estimation/Velocity from vehicle body frame to inertial NED  frame ==
  data: Vel_b input; Vel_xy output; psi input
function Vel_xy = fcn(Vel_b , psi)
%#codegen
T = [cos(psi) -sin(psi) ; sin(psi) cos(psi)] ; 
Vel_xy = T*Vel_b(1:2,1);

== matlab function ARDroneControl/Baseline Controller/Heading controller/normalize angle between -pi and pi radians ==
  data: angleIn input; angleOut output
function angleOut = fcn(angleIn)
%#codegen

angleOut = mod(angleIn, 2*pi) ;
if angleOut > pi
    angleOut = -2*pi + angleOut ; 
end

== matlab function ARDroneControl/MATLAB Function2 ==
  data: bw input; Z output
function Z = distance_estimation(bw)
% Distance estimation based on Pinhole model

% Constants 
%fu = 562.88; % Horizontal focal length [px]
fu = 562.88;
W = 0.288; % Minimum object width [m]

% Inputs
% bw = bounding box width

Z = fu*W/bw;

== matlab function ARDroneControl/MATLAB Function3 ==
  data: s input; e input; Vc output
function Vc = ibvs_controller(s,e)

l1 = 0.001;
l2 = -1;
l3 = 0.28; %0.095 ultimo test 21-09-2026 17:56
l4 = 0.001;
l5 = 0.25; %0.92
l6 = 0.001;

Lambda = diag([l1 l2 l3 l4 l5 l6]);

x = s(1);
y = s(2);
Z = s(3);

Le = [-1/Z, 0, x/Z, x*y, -(1+x^2), y;
      0, -1/Z, y/Z, 1+y^2, -x*y, -x;
      0, 0, -1, -y*Z, x*Z, 0];

% x,y ideal = 0
%Z_star = Z;
Z_star = 1;
Le_star = [-1/Z_star, 0, 0, 0, -1, 0;
            0, -1/Z_star, 0, 1, 0, 0;
            0, 0, -1, 0, 0, 0];

Le_pseudoinver = 0.5*pinv(Le+Le_star);

e = e(:); % Column vector

Vc = -Lambda*Le_pseudoinver*e;

== matlab function ARDroneControl/Subsystem1/MATLAB Function1 ==
  data: Z input; Kp output
function Kp = yaw_decay_gain(Z)

    M = 0.03;
    Z_star = 0;

    sigma = sqrt(((-0.5)^1)/log(0.66));

    Kp = M*(1-exp(-0.5*((Z-Z_star)/sigma)^2));

end
